simulink model "hrg_wa_v5_envelope"  (R2025a)
settings: Solver=ode4  StartTime=0.0  StopTime=wl_stop  FixedStep=wl_Tc  RelTol=1e-3
PostLoadFcn:
  | addpath(fileparts(fileparts(get_param('hrg_wa_v5_envelope','FileName')))); wl_setup(getVariable(get_param('hrg_wa_v5_envelope','ModelWorkspace'),'wl_saved_configuration'));
model workspace (MAT data in the model file):
  wl_saved_configuration.stage = 5
  wl_saved_configuration.name = 'hrg_wa_v5'
  wl_saved_configuration.head.sourceProfile = 'C:\Users\11725\Desktop\HRG_WA\HRG_WA_simulink\..\HRG_WA_Digital_ASIC_MATLAB_v4_6_5_FRP_validation_fix\HRG_WA\config\head_default.json'
  wl_saved_configuration.head.measurementStatus = 'assumed, not a measured head'
  wl_saved_configuration.head.f0 = 5000
  wl_saved_configuration.head.Q = 2000000
  wl_saved_configuration.head.bryan = 0.277
  wl_saved_configuration.head.gamma = 0.00785398163397
  wl_saved_configuration.head.dgamma = 0.00025
  wl_saved_configuration.head.dampingAxis = 0.296705972839
  wl_saved_configuration.head.splitHz = 0.008
  wl_saved_configuration.head.stiffnessAxis = 0.715584993318
  wl_saved_configuration.head.detuningHz = 0
  wl_saved_configuration.head.duffingHz = 0.015
  wl_saved_configuration.head.temperatureCoeff = -1.8e-05
  wl_saved_configuration.head.referenceTemperature = 25
  wl_saved_configuration.head.detect = [1  0.003; -0.002  1]
  wl_saved_configuration.head.detectPhase = [0; 0]
  wl_saved_configuration.head.drive = [1  0; 0  1]
  wl_saved_configuration.head.detectCubic = 0
  wl_saved_configuration.head.iqBits = 0
  wl_saved_configuration.head.iqFullScale = 2
  wl_saved_configuration.head.energyTarget = 1
  wl_saved_configuration.head.initialEnergy = 1
  wl_saved_configuration.head.initialTheta = 0.13962634016
  wl_saved_configuration.head.initialQuadRatio = 0
  wl_saved_configuration.head.energyKp = 0.8
  wl_saved_configuration.head.energyKi = 0.4
  wl_saved_configuration.head.quadKp = 2
  wl_saved_configuration.head.quadKi = 1
  wl_saved_configuration.head.pllKp = 0.8
  wl_saved_configuration.head.pllKi = 1
  wl_saved_configuration.head.energyLimit = 1
  wl_saved_configuration.head.quadLimit = 1
  wl_saved_configuration.head.pllLimitHz = 2
  wl_saved_configuration.head.antiWindup = 5
  wl_saved_configuration.head.loopEnable = 1
  wl_saved_configuration.head.Ts = 0.001
  wl_saved_configuration.head.rateTau = 0.00353677651315
  wl_saved_configuration.head.energyThreshold = 0.02
  wl_saved_configuration.head.angleThreshold = 0.01
  wl_saved_configuration.head.duration = 12
  wl_saved_configuration.head.omega = 1.3962634016
  wl_saved_configuration.head.virtualRate = 0
  wl_saved_configuration.head.temperature = 25
  wl_saved_configuration.head.fullStep = 2e-06
  wl_saved_configuration.fsAdc = 40000
  wl_saved_configuration.fsPlant = 400000
  wl_saved_configuration.duration = 1
  wl_saved_configuration.seed = 20261021
  wl_saved_configuration.massKg = 1e-06
  wl_saved_configuration.displacementM = 1e-07
  wl_saved_configuration.gapM = 5e-06
  wl_saved_configuration.c0F = 1e-12
  wl_saved_configuration.cfF = 1e-12
  wl_saved_configuration.rfOhm = 1000000000
  wl_saved_configuration.biasV = 10
  wl_saved_configuration.cvBandwidthHz = 30000
  wl_saved_configuration.pgaBandwidthHz = 30000
  wl_saved_configuration.pgaGain = 1
  wl_saved_configuration.cvEnVrtHz = 1e-08
  wl_saved_configuration.cvInArtHz = 1e-14
  wl_saved_configuration.temperatureK = 298.15
  wl_saved_configuration.pgaNoiseVrtHz = 1e-08
  wl_saved_configuration.afeOffsetV = [0; 0]
  wl_saved_configuration.afeLimitV = 1.8
  wl_saved_configuration.adcBits = 18
  wl_saved_configuration.adcFsV = 2
  wl_saved_configuration.adcOffsetV = [0; 0]
  wl_saved_configuration.adcGain = [1; 1]
  wl_saved_configuration.adcInlCubic = 0
  wl_saved_configuration.jitterRmsS = 2e-09
  wl_saved_configuration.channelSkewS = 0
  wl_saved_configuration.adcDelay = 1
  wl_saved_configuration.adcArchitecture = 'nyquist'
  wl_saved_configuration.cicStages = 3
  wl_saved_configuration.fir = [0.111111111111 0.222222222222 0.333333333333 0.222222222222 0.111111111111]
  wl_saved_configuration.dacBits = 16
  wl_saved_configuration.dacFsV = 2
  wl_saved_configuration.dacDelay = 1
  wl_saved_configuration.dacInlCubic = 0
  wl_saved_configuration.dacArchitecture = 'nyquist'
  wl_saved_configuration.driveNPerV = 1e-07
  wl_saved_configuration.driverBandwidthHz = 50000
  wl_saved_configuration.driverGain = [1; 1]
  wl_saved_configuration.driverSlewVPerS = 200000
  wl_saved_configuration.driverNoiseVrtHz = 2e-08
  wl_saved_configuration.driverLimitV = 1.8
  wl_saved_configuration.feedthroughF = 0
  wl_saved_configuration.pipelineCtrl = 3
  wl_saved_configuration.iqFractionBits = 22
  wl_saved_configuration.controlFractionBits = 22
  wl_saved_configuration.antiAliasHz = 18000
  wl_saved_configuration.noiseEnable = 1
  wl_saved_configuration.circuitEnable = 1
  wl_saved_configuration.kalman = 1
  wl_saved_configuration.online = 0
  wl_saved_configuration.frp = 0
  wl_saved_configuration.calibrationPermit = 0
  wl_saved_configuration.frpSequence = 0
  wl_saved_configuration.frpFreeze = 0
  wl_saved_configuration.frpTheta = [0; 0; 0; 0; 0; 0; 0; 0; 0]
  wl_saved_configuration.matrixApply = 0
  wl_saved_configuration.compensationApply = 0
  wl_saved_configuration.temperatureCompensate = 0
  wl_saved_configuration.temperatureBiasCoefficients = [0; 0; 0]
  wl_saved_configuration.zeroRateCertified = 0
  wl_saved_configuration.virtualRate = 0
  wl_saved_configuration.inputRate = 1.3962634016
  wl_saved_configuration.inputFrequencyHz = 0
  wl_saved_configuration.inputRateAmplitude = 0
  wl_saved_configuration.temperatureC = 25
  wl_saved_configuration.temperatureRampCPerS = 0
  wl_saved_configuration.observers = 1
  wl_saved_configuration.spectra = 1
  wl_saved_configuration.maxLogPoints = 80000
  wl_saved_configuration.sdmLeak = 0.9999
  wl_saved_configuration.sdmReferenceV = 2
  wl_saved_configuration.tdmEnable = 0
  wl_saved_configuration.knownPhaseCalibrationRad = -2.63258802151
  wl_saved_configuration.virtualGainCalibration = 1.10062721786
  wl_saved_configuration.learnStartS = 0.25
  wl_saved_configuration.measurementStatus = 'assumed'
  wl_saved_configuration.scope = 'Behavioral circuit interfaces, not transistor or bit-true RTL signoff'
  wl_saved_configuration.cvEquivalentNoiseVrtHz = 3.43925722091e-07
undefined symbols (not defined in the file): wa_plant_rhs, wl_c, wl_control_tick, wl_detectGain, wl_env_adc, wl_env_drive, wl_env_noise, wl_env_sense, wl_env_z0, wl_fir, wl_input, wl_iq_quantize, wl_p, wl_Tc
settings Model: Creator=11725  LastModifiedBy=11725
settings DataIOCC: SaveOutput=off
settings DebuggingCC: AlgebraicLoopMsg=error

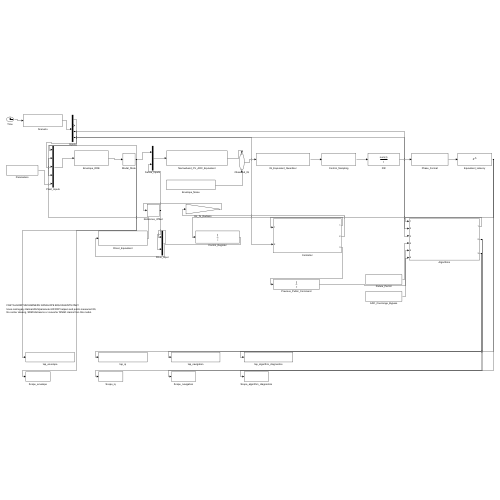
[thumbnail: Simulink's stored preview of the top-level diagram]
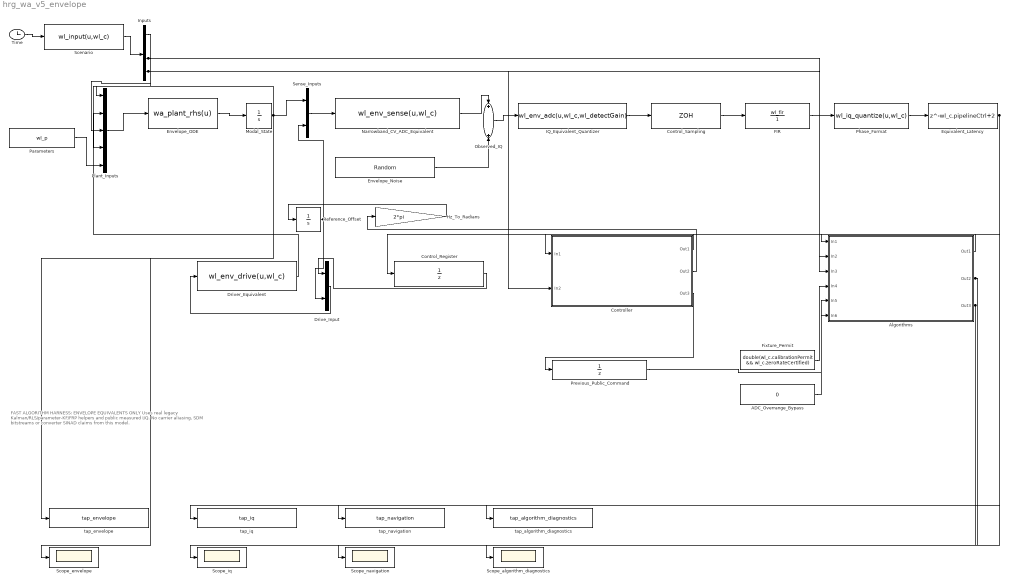
== system hrg_wa_v5_envelope ==
  note: FAST ALGORITHM HARNESS: ENVELOPE EQUIVALENTS ONLY
      | Uses real legacy Kalman/RLS/parameter-KF/FRP helpers and public measured I/Q.
      | No carrier aliasing, SDM bitstreams or converter SINAD claims from this model.
  ADC_Overrange_Bypass : Constant  Value=0
  Algorithms : Subsystem
  Control_Register : UnitDelay  InitialCondition=zeros(4,1)  SampleTime=wl_Tc  HasFrameUpgradeWarning=on
  Control_Sampling : ZeroOrderHold  SampleTime=wl_Tc
  Controller : Subsystem
  Drive_Input : Mux  Inputs=2
  Driver_Equivalent : MATLABFcn  MATLABFcn=wl_env_drive(u,wl_c)  OutputDimensions=4
  Envelope_Noise : RandomNumber  Mean=zeros(4,1)  Variance=wl_env_noise*ones(4,1)  Seed=wl_c.seed+[701;702;703;704]  SampleTime=wl_Tc
  Envelope_ODE : MATLABFcn  MATLABFcn=wa_plant_rhs(u)  OutputDimensions=4
  Equivalent_Latency : Delay  DelayLength=wl_c.pipelineCtrl+2  InitialCondition=0  SampleTime=wl_Tc
  FIR : DiscreteFilter  Numerator=wl_fir  Denominator=1  SampleTime=wl_Tc
  Fixture_Permit : Constant  Value=double(wl_c.calibrationPermit && wl_c.zeroRateCertified)
  Hz_To_Radians : Gain  Gain=2*pi
  IQ_Equivalent_Quantizer : MATLABFcn  MATLABFcn=wl_env_adc(u,wl_c,wl_detectGain)  OutputDimensions=4
  Inputs : Demux  Outputs=[1 1 1 1]
  Modal_State : Integrator  InitialCondition=wl_env_z0
  Narrowband_CV_ADC_Equivalent : MATLABFcn  MATLABFcn=wl_env_sense(u,wl_c)  OutputDimensions=4
  Observed_IQ : Sum
  Parameters : Constant  Value=wl_p
  Phase_Format : MATLABFcn  MATLABFcn=wl_iq_quantize(u,wl_c)  OutputDimensions=4
  Plant_Inputs : Mux  Inputs=5
  Previous_Public_Command : UnitDelay  InitialCondition=zeros(3,1)  SampleTime=wl_Tc  HasFrameUpgradeWarning=on
  Reference_Offset : Integrator
  Scenario : MATLABFcn  MATLABFcn=wl_input(u,wl_c)  OutputDimensions=4
  Scope_algorithm_diagnostics : Scope
  Scope_envelope : Scope
  Scope_iq : Scope
  Scope_navigation : Scope
  Sense_Inputs : Mux  Inputs=2
  Time : Clock
  tap_algorithm_diagnostics : ToWorkspace  VariableName=tap_algorithm_diagnostics  SaveFormat=Timeseries  SampleTime=-1
  tap_envelope : ToWorkspace  VariableName=tap_envelope  SaveFormat=Timeseries  SampleTime=-1
  tap_iq : ToWorkspace  VariableName=tap_iq  SaveFormat=Timeseries  SampleTime=-1
  tap_navigation : ToWorkspace  VariableName=tap_navigation  SaveFormat=Timeseries  SampleTime=-1
  wires:
  Time/1 -> Scenario/1
  Scenario/1 -> Inputs/1
  Modal_State/1 -> Plant_Inputs/1, Sense_Inputs/1, tap_envelope/1, Scope_envelope/1
  Inputs/1 -> Plant_Inputs/3
  Inputs/3 -> Plant_Inputs/4, Algorithms/2(In2)
  Parameters/1 -> Plant_Inputs/5
  Plant_Inputs/1 -> Envelope_ODE/1
  Envelope_ODE/1 -> Modal_State/1
  Reference_Offset/1 -> Sense_Inputs/2, Drive_Input/2
  Sense_Inputs/1 -> Narrowband_CV_ADC_Equivalent/1
  Narrowband_CV_ADC_Equivalent/1 -> Observed_IQ/1
  Envelope_Noise/1 -> Observed_IQ/2
  Observed_IQ/1 -> IQ_Equivalent_Quantizer/1
  IQ_Equivalent_Quantizer/1 -> Control_Sampling/1
  Control_Sampling/1 -> FIR/1
  FIR/1 -> Phase_Format/1
  Phase_Format/1 -> Equivalent_Latency/1
  Equivalent_Latency/1 -> Algorithms/1(In1), tap_iq/1, Scope_iq/1
  Inputs/4 -> Algorithms/3(In3), Controller/2(In2)
  Fixture_Permit/1 -> Algorithms/4(In4)
  Previous_Public_Command/1 -> Algorithms/5(In5)
  ADC_Overrange_Bypass/1 -> Algorithms/6(In6)
  Algorithms/1(Out1) -> Controller/1(In1)
  Controller/3(Out3) -> Previous_Public_Command/1
  Controller/1(Out1) -> Control_Register/1
  Control_Register/1 -> Drive_Input/1
  Drive_Input/1 -> Driver_Equivalent/1
  Driver_Equivalent/1 -> Plant_Inputs/2
  Controller/2(Out2) -> Hz_To_Radians/1
  Hz_To_Radians/1 -> Reference_Offset/1
  Algorithms/2(Out2) -> tap_navigation/1, Scope_navigation/1
  Algorithms/3(Out3) -> tap_algorithm_diagnostics/1, Scope_algorithm_diagnostics/1

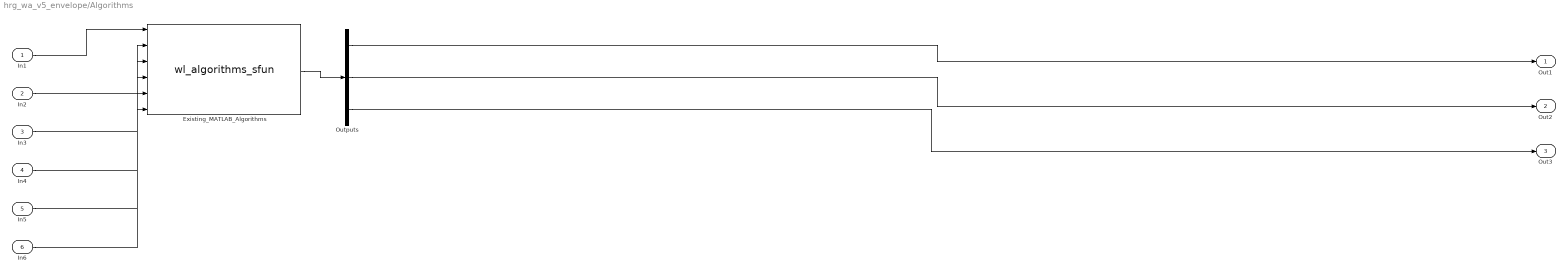
== system hrg_wa_v5_envelope/Algorithms ==
  In1 : Inport
  In2 : Inport  Port=2
  In3 : Inport  Port=3
  In4 : Inport  Port=4
  In5 : Inport  Port=5
  In6 : Inport  Port=6
  Existing_MATLAB_Algorithms : M-S-Function  FunctionName=wl_algorithms_sfun  Parameters=wl_c
  Outputs : Demux  Outputs=[10 4 21]
  Out1 : Outport
  Out2 : Outport  Port=2
  Out3 : Outport  Port=3
  wires:
  Outputs/3 -> Out3/1
  Outputs/2 -> Out2/1
  Outputs/1 -> Out1/1
  Existing_MATLAB_Algorithms/1 -> Outputs/1
  In6/1 -> Existing_MATLAB_Algorithms/6
  In5/1 -> Existing_MATLAB_Algorithms/5
  In4/1 -> Existing_MATLAB_Algorithms/4
  In3/1 -> Existing_MATLAB_Algorithms/3
  In2/1 -> Existing_MATLAB_Algorithms/2
  In1/1 -> Existing_MATLAB_Algorithms/1

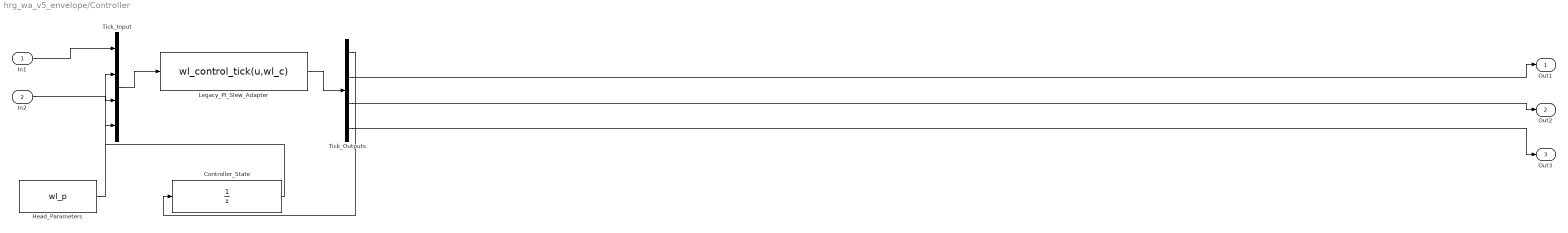
== system hrg_wa_v5_envelope/Controller ==
  In1 : Inport
  In2 : Inport  Port=2
  Controller_State : UnitDelay  InitialCondition=zeros(6,1)  SampleTime=wl_Tc  HasFrameUpgradeWarning=on
  Head_Parameters : Constant  Value=wl_p
  Legacy_PI_Slew_Adapter : MATLABFcn  MATLABFcn=wl_control_tick(u,wl_c)  OutputDimensions=14
  Tick_Input : Mux
  Tick_Outputs : Demux  Outputs=[6 4 1 3]
  Out1 : Outport
  Out2 : Outport  Port=2
  Out3 : Outport  Port=3
  wires:
  Tick_Outputs/4 -> Out3/1
  Tick_Outputs/3 -> Out2/1
  Tick_Outputs/2 -> Out1/1
  Tick_Outputs/1 -> Controller_State/1
  Legacy_PI_Slew_Adapter/1 -> Tick_Outputs/1
  Tick_Input/1 -> Legacy_PI_Slew_Adapter/1
  Head_Parameters/1 -> Tick_Input/4
  In2/1 -> Tick_Input/3
  Controller_State/1 -> Tick_Input/2
  In1/1 -> Tick_Input/1
